simulink model "LQG_linear_sim"  (R2026a)
settings: Solver=VariableStepAuto
InitFcn:
  | actuator = actuator_params_nominal();
  | [Gact, info] = build_nominal_actuator(actuator);
  | 
  | % Parametri del robot
  | p = sea_params_nominal();
  | Simulink.Bus.createObject(p);
  | 
  | % Equilibrio desiderato
  | qbar = [pi/2; 0];
  | 
  | % Calcolo stato e coppia di equilibrio
  | [xbar, taubar, info] = sea_static_equilibrium(qbar, p);
  | 
  | 
  | 
  | %% INITFCN - Pianta LQGI lineare a 14 stati con 8 ingressi
  | 
  | % Individua la root del progetto partendo da progetto_lqgi.m
  | projectFile = which('progetto_lqgi.m');
  | 
  | assert(~isempty(projectFile), ...
  |     ['progetto_lqgi.m non trovato. Eseguire prima lo script ' ...
  |     'e verificare il MATLAB path.']);
  | 
  | projectRoot = fileparts(fileparts(projectFile));
  | dataDir = fullfile(projectRoot, 'results', 'data');
  | 
  | % File prodotti dagli script di validazione M3 e M5
  | m3File = fullfile(dataDir, 'm3_nominal_actuated_plant.mat');
  | m5File = fullfile(dataDir, 'm5_performance_specs.mat');
  | 
  | % Verifica che i dati della pianta esistano
  | assert(isfile(m3File), ...
  |     'Manca m3_nominal_actuated_plant.mat. Eseguire la validazione M3.');
  | 
  | % Se M5 non e' ancora stato generato, costruisce BdFull
  | if ~isfile(m5File)
  |     addpath(genpath(fullfile(projectRoot, 'src')));
  |     addpath(genpath(fullfile(projectRoot, 'analysis')));
  |     validate_m5_performance_specs;
  | end
  | 
  | assert(isfile(m5File), ...
  |     'Manca m5_performance_specs.mat dopo la validazione M5.');
  | 
  | % Carica le matrici necessarie
  | m3 = load(m3File, 'Afull', 'Bfull', 'CfullMeas');
  | m5 = load(m5File, 'BdFull');
  | 
  | Aplant = m3.Afull;
  | Bfull = m3.Bfull;
  | BdFull = m5.BdFull;
  | Cplant = m3.CfullMeas;
  | 
  | % Controlli sulle dimensioni delle matrici
  | assert(isequal(size(Aplant), [14 14]));
  | assert(isequal(size(Bfull), [14 2]));
  | assert(isequal(size(BdFull), [14 2]));
  | assert(isequal(size(Cplant), [4 14]));
  | 
  | % Ordine degli ingressi:
  | % 1-2: comando u
  | % 3-4: disturbo deterministico d lato link
  | % 5-6: rumore di processo w_link
  | % 7-8: rumore di processo w_u lato ingresso
  | 
  | Bplant = [Bfull, BdFull, BdFull, Bfull];
  | 
  | % Nessuna trasmissione diretta dagli ingressi alle misure
  | Dplant = zeros(4, 8);
  | 
  | % Condizione iniziale del modello linearizzato in deviazioni
  | x0plant = zeros(14, 1);
  | 
  | % Pubblica le variabili nel Base Workspace per i blocchi Simulink
  | assignin('base', 'Aplant', Aplant);
  | assignin('base', 'Bplant', Bplant);
  | assignin('base', 'Cplant', Cplant);
  | assignin('base', 'Dplant', Dplant);
  | assignin('base', 'x0plant', x0plant);
  | 
  | % Mantiene disponibili anche le matrici originali
  | assignin('base', 'Afull', Aplant);
  | assignin('base', 'Bfull', Bfull);
  | assignin('base', 'BdFull', BdFull);
  | assignin('base', 'CfullMeas', Cplant);
  | 
  | fprintf(['InitFcn LQGI: Aplant %dx%d, Bplant %dx%d, ' ...
  |     'Cplant %dx%d, Dplant %dx%d.\\n'], ...
  |     size(Aplant,1), size(Aplant,2), ...
  |     size(Bplant,1), size(Bplant,2), ...
  |     size(Cplant,1), size(Cplant,2), ...
  |     size(Dplant,1), size(Dplant,2));
undefined symbols (not defined in the file): A, B, C, K, L, Nr
settings Model: Creator=rebec  LastModifiedBy=rebec

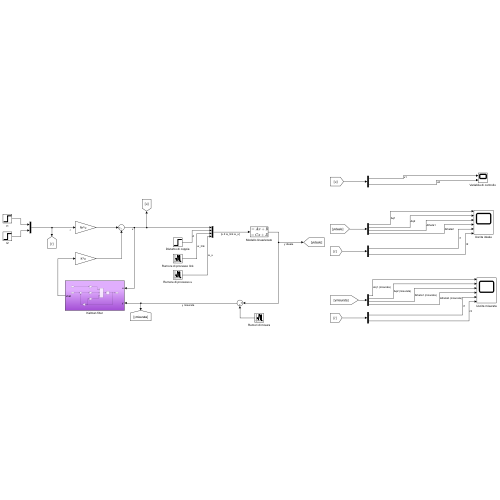
[thumbnail: Simulink's stored preview of the top-level diagram]
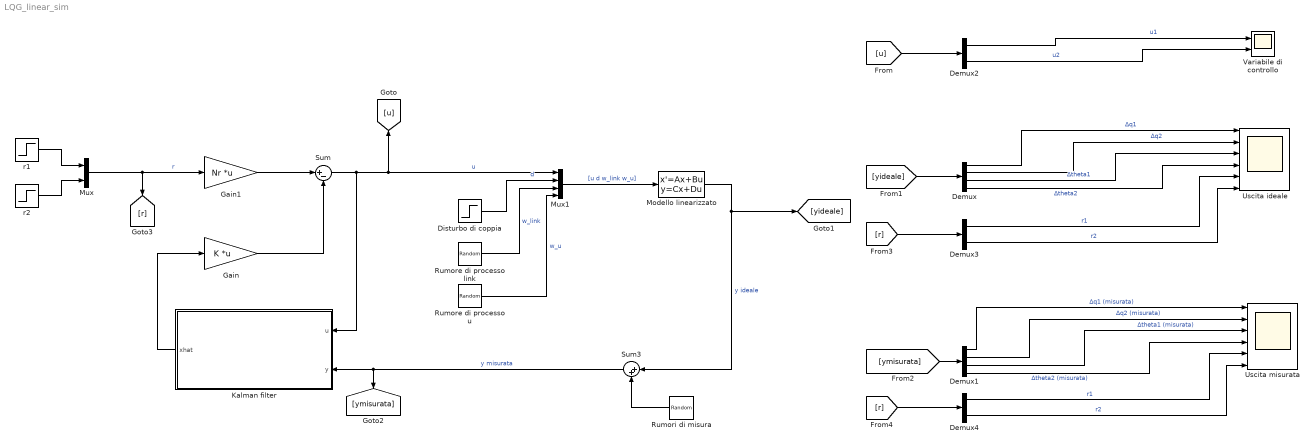
== system LQG_linear_sim ==
  Demux : Demux
  Demux1 : Demux
  Demux2 : Demux  Outputs=2
  Demux3 : Demux  Outputs=2
  Demux4 : Demux  Outputs=2
  Disturbo di coppia : Step  Time=[1 1]  InitialValue=[0 0]  FinalValue=[0.5 0]  SampleTime=0
  Gain : Gain  Gain=K  Multiplication=Matrix(K*u)
  Gain1 : Gain  Gain=Nr  Multiplication=Matrix(K*u)
  Kalman filter : Subsystem
  Modello linearizzato : StateSpace  A=Aplant  B=Bplant  C=Cplant  D=Dplant  InitialCondition=x0plant
  Mux : Mux  Inputs=2
  Mux1 : Mux
  Rumore di processo link : RandomNumber  Mean=[0 0]  Variance=[0.01 0.01]  Seed=20260826  SampleTime=0.002
  Rumore di processo u : RandomNumber  Mean=[0 0]  Variance=[0.01 0.01]  Seed=20260826  SampleTime=0.002
  Rumori di misura : RandomNumber  Mean=[0 0 0 0]  Variance=[(0.05*pi/180)^2 (0.05*pi/180)^2 (0.05*pi/180)^2 (0.05*pi/180)^2]  Seed=20260826  SampleTime=0.002
  Sum : Sum  Inputs=|+-
  Sum3 : Sum  Inputs=|++
  Uscita ideale : Scope  NumInputPorts=6
      settings: Title=y (uscita ideale)  ActiveDisplayYMinimum=-0.094752290571448711  ActiveDisplayYMaximum=0.25948345010826868
  Uscita misurata : Scope  NumInputPorts=6
      settings: Title=y (uscita ideale)  ActiveDisplayYMinimum=-0.11442029066688837  ActiveDisplayYMaximum=0.16914890182413583
  Variabile di controllo : Scope  NumInputPorts=2
      settings: ActiveDisplayYMinimum=-2.6959450601265313  ActiveDisplayYMaximum=5.9059369724787079  DataLoggingVariableName=ScopeData2
  r1 : Step  FinalValue=5*pi/180  SampleTime=0
  r2 : Step  FinalValue=0  SampleTime=0
  wires:
  Demux/4 -> Uscita ideale/4  "Δtheta2"
  Demux2/1 -> Variabile di controllo/1  "u1"
  Demux1/1 -> Uscita misurata/1  "Δq1 (misurata)"
  r2/1 -> Mux/2
  Demux1/4 -> Uscita misurata/4  "Δtheta2 (misurata)"
  [r] -> Demux3/1
  Demux1/3 -> Uscita misurata/3  "Δtheta1 (misurata)"
  [u] -> Demux2/1
  [ymisurata] -> Demux1/1
  Demux3/1 -> Uscita ideale/5  "r1"
  Demux/1 -> Uscita ideale/1  "Δq1"
  Demux4/1 -> Uscita misurata/5  "r1"
  Demux1/2 -> Uscita misurata/2  "Δq2 (misurata)"
  Modello linearizzato/1 -> Sum3/1, [yideale]  "y ideale"
  Sum3/1 -> [ymisurata], Kalman filter/2(y)  "y misurata"
  r1/1 -> Mux/1
  Gain1/1 -> Sum/1
  [yideale] -> Demux/1
  Demux2/2 -> Variabile di controllo/2  "u2"
  Demux/2 -> Uscita ideale/2  "Δq2"
  Demux/3 -> Uscita ideale/3  "Δtheta1"
  Demux3/2 -> Uscita ideale/6  "r2"
  Sum/1 -> Mux1/1, [u], Kalman filter/1(u)  "u"
  Demux4/2 -> Uscita misurata/6  "r2"
  Mux/1 -> [r], Gain1/1  "r"
  [r] -> Demux4/1
  Kalman filter/1(xhat) -> Gain/1
  Gain/1 -> Sum/2
  Rumore di processo u/1 -> Mux1/4  "w_u"
  Disturbo di coppia/1 -> Mux1/2  "d"
  Rumore di processo link/1 -> Mux1/3  "w_link"
  Mux1/1 -> Modello linearizzato/1  "[u d w_link w_u]"
  Rumori di misura/1 -> Sum3/2

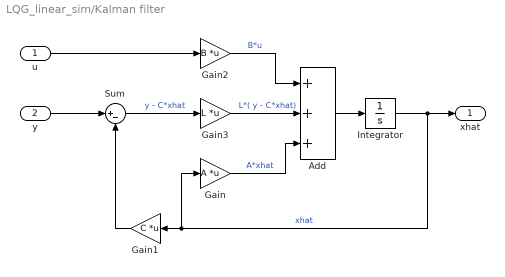
== system LQG_linear_sim/Kalman filter ==
  u : Inport
  y : Inport  Port=2
  Add : Sum  Inputs=+++
  Gain : Gain  Gain=A  Multiplication=Matrix(K*u)
  Gain1 : Gain  Gain=C  Multiplication=Matrix(K*u)
  Gain2 : Gain  Gain=B  Multiplication=Matrix(K*u)
  Gain3 : Gain  Gain=L  Multiplication=Matrix(K*u)
  Integrator : Integrator
  Sum : Sum  Inputs=|+-
  xhat : Outport
  wires:
  u/1 -> Gain2/1
  y/1 -> Sum/1
  Gain1/1 -> Sum/2
  Sum/1 -> Gain3/1  "y - C*xhat"
  Gain3/1 -> Add/2  "L*( y - C*xhat)"
  Gain2/1 -> Add/1  "B*u"
  Gain/1 -> Add/3  "A*xhat"
  Add/1 -> Integrator/1
  Integrator/1 -> Gain/1, Gain1/1, xhat/1  "xhat"
